simulink model "buck"  (R2026a)
settings: Solver=ode23t  StopTime=simlength  FixedStep=tc  MaxStep=glb_time.tc  RelTol=1e-4
values from neighbouring files (symbols this model uses):
  afe_pwm_phase_shift_mod1 = 0    [init_model.m]
  glb_time = timing_setup(fpwm_afe, trgo_afe, fpwm_inv, trgo_inv, fpwm_single_phase_inv, trgo_single_phase_inv, fpwm_dab, trgo_dab,      fpwm_psfbc, trgo_psfbc, fpwm_isop_rail, trgo_isop_rail, fpwm_cllc, trgo_cllc, t_measure, tc_factor, tc_decimation, delay_pwm, dead_time_afe,      dead_time_inv, dead_time_single_phase_inv, dead_time_dab, dead_time_psfbc, dead_time_isop_rail, dead_time_cllc)    [init_model.m]
  time_gain_afe_module_1 = 1.0002    [init_model.m]
  time_gain_inv_module_2 = 1.001    [init_model.m]
libraries: fl_lib x23, nesl_utility x14, diode_rr_lib x2, igbt_dyn_lib x2, ee_lib x1, dclink_for_two_levels x1, single_phase_pwm_modulator x1
(part 2 of 2)

== system buck/buck/leg/leg/leg_with_igbt_dyn/leg_with_igbt_dyn/igbt_dyn_2/IGBT_dyn/IGBT_dyn/IGBT_dyn/igbt_dyn ==
  IGBT (switching dynamics) : igbt_dyn_lib/IGBT (switching dynamics)  Vth=6.5 V  Kp=100 A/V^2  lam=0 1/V  Cge=180e-9 F  Cgc0=25e-9 F  Vjc=1 V  mc=0.7  Cce0=30e-9 F  Vjo=1 V  mo=0.5  Rg=1 Ohm  ftail=0.25  tauT=1.5e-6 s  dsm=0.5 V  ig_specify=off  ig_priority=None  ig=0 A  ig_nominal_specify=off  ig_nominal_value=1  ig_nominal_unit=A  ige_specify=off  ige_priority=None  ige=0 A  ige_nominal_specify=off  ige_nominal_value=1  ige_nominal_unit=A  igc_specify=off  igc_priority=None  igc=0 A  igc_nominal_specify=off  igc_nominal_value=1  igc_nominal_unit=A  ich_specify=off  ich_priority=None  ich=0 A  ich_nominal_specify=off  ich_nominal_value=1  ich_nominal_unit=A  icap_specify=off  icap_priority=None  icap=0 A  icap_nominal_specify=off  icap_nominal_value=1  icap_nominal_unit=A  itl_specify=off  itl_priority=None  itl=0 A  itl_nominal_specify=off  itl_nominal_value=1  itl_nominal_unit=A  vge_specify=off  vge_priority=None  vge=0 V  vge_nominal_specify=off  vge_nominal_value=1  vge_nominal_unit=V  vgc_specify=off  vgc_priority=None  vgc=0 V  vgc_nominal_specify=off  vgc_nominal_value=1  vgc_nominal_unit=V  vce_specify=off  vce_priority=None  vce=10 V  vce_nominal_specify=off  vce_nominal_value=1  vce_nominal_unit=V  qge_specify=off  qge_priority=None  qge=0 C  qge_nominal_specify=off  qge_nominal_value=1  qge_nominal_unit=C  qgc_specify=off  qgc_priority=None  qgc=0 C  qgc_nominal_specify=off  qgc_nominal_value=1  qgc_nominal_unit=C  qce_specify=off  qce_priority=None  qce=0 C  qce_nominal_specify=off  qce_nominal_value=1  qce_nominal_unit=C
  G : PMIOPort  Side=Left
  C : PMIOPort  Port=2  Side=Left
  E : PMIOPort  Port=3  Side=Right
  connections:
  IGBT (switching dynamics)/RConn1 -- C/RConn1
  IGBT (switching dynamics)/LConn1 -- G/RConn1
  IGBT (switching dynamics)/RConn2 -- E/RConn1

== matlab function buck/leg/leg/leg_pwm/modulator1/one phase PWM generator with global TRGO/MATLAB Function ==
  data: t input; y output; phase input; period input
function y = ramp_up_down(t,phase,period)
x = sin(2*pi/period*t - phase -pi/2);
y = asin(x)/pi + 1/2;
